simulink model "GFM_Controller_C"  (R2025b)
settings: Solver=VariableStepAuto  StartTime=0.0  StopTime=10.0  RelTol=1e-3
values from neighbouring files (symbols this model uses):
  a = 0.5    [GFM_Simulink_Init_GUI_v3.m]
  b = (beta*gamma)/(beta + gamma - a)    [GFM_Simulink_Init_GUI_v3.m]
  c = (beta + gamma - a)/mp    [GFM_Simulink_Init_GUI_v3.m]
  D1 = Moh_Dp/Moh_Sbase    (= 0.2546)    [GFM_Simulink_Init_GUI_v3.m]
  D2 = 0.4    [GFM_Simulink_Init_GUI_v3.m]
  delta2_0 = delta2PCC0 + atan2(      Pm2_0*X2/V2PCCmag0,      V2PCCmag0 + Q21_0*X2/V2PCCmag0 )    [GFM_Simulink_Init_GUI_v3.m]
  Dw2_0 = 0    [GFM_Simulink_Init_GUI_v3.m]
  E2_0 = hypot(      Pm2_0*X2/V2PCCmag0,      V2PCCmag0 + Q21_0*X2/V2PCCmag0 )    [GFM_Simulink_Init_GUI_v3.m]
  H2 = 12    [GFM_Simulink_Init_GUI_v3.m]
  Imax = 1.20    (= 1.2)    [GFM_Simulink_Init_GUI_v3.m]
  Ki = 0.5    [GFM_Simulink_Init_GUI_v3.m]
  Kiq = Moh_Kiq*Moh_Sbase/Moh_Vbase    [GFM_Simulink_Init_GUI_v3.m]
  Lf = 1e-3    (= 0.001)    [GFM_Simulink_Init_GUI_v3.m]
  LimitEnable = 0    [GFM_Simulink_Init_GUI_v3.m]
  Ls = Xs/ws    [GFM_Simulink_Init_GUI_v3.m]
  nq = Moh_nq*Moh_Sbase/Moh_Vbase    [GFM_Simulink_Init_GUI_v3.m]
  Pload_0 = P12_0    (= 1)    [GFM_Simulink_Init_GUI_v3.m]
  Qref = 0.0    (= 0)    [GFM_Simulink_Init_GUI_v3.m]
  Rf = 1.0    (= 1)    [GFM_Simulink_Init_GUI_v3.m]
  RLFault = 0    [GFM_Simulink_Init_GUI_v3.m]
  Rs = Zs_mag/sqrt(1 + XR_grid^2)    [GFM_Simulink_Init_GUI_v3.m]
  SolidFault = 0    [GFM_Simulink_Init_GUI_v3.m]
  ws = 2*pi*f    (= 314.159265359)    [GFM_Simulink_Init_GUI_v3.m]
  X1 = Xtf_src_total_pu    (= 0.15)    [GFM_Simulink_Init_GUI_v3.m]
libraries: nesl_utility x12, ee_lib x11, fl_lib x6, eePowerMeasurement x1
settings Model: Creator=Nicholas  LastModifiedBy=Nicholas

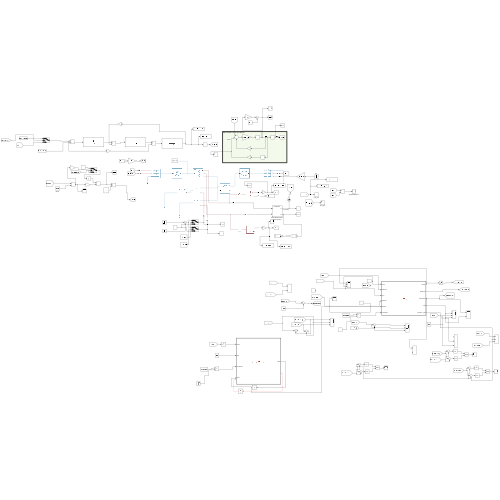
[thumbnail: Simulink's stored preview of the top-level diagram]
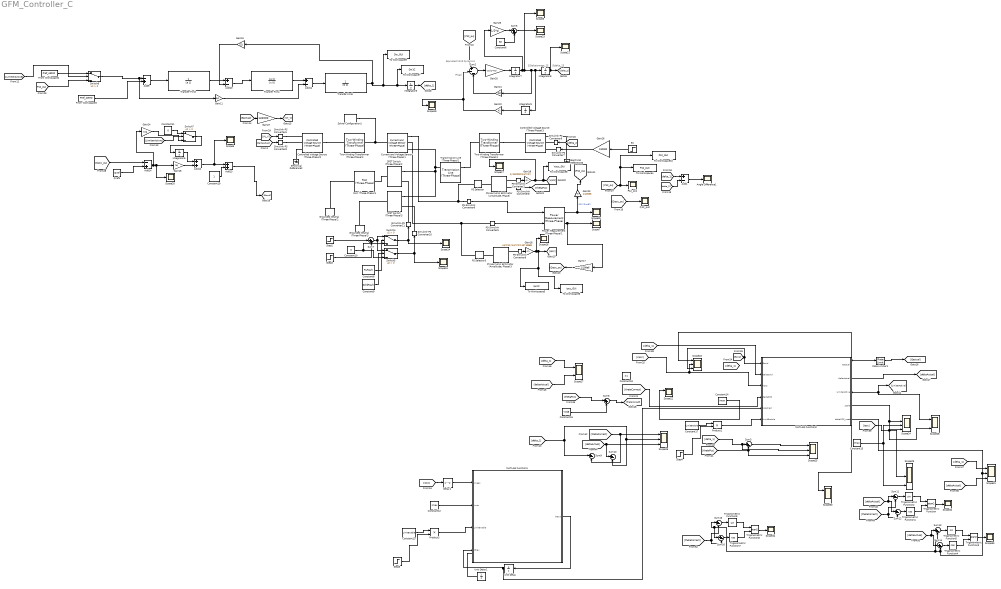
== system GFM_Controller_C ==
  note: $\delta_2$
  note: Pload
  note: $\Delta\omega_2$
  note: Equivalent Grid Dynamics
  Add1 : Sum  Inputs=+-
  Add10 : Sum  Inputs=+-
  Add11 : Sum  Inputs=+-
  Add12 : Sum
  Add13 : Sum
  Add14 : Sum  Inputs=-+
  Add9 : Sum  Inputs=-+
  Angle Difference1 : Scope
      settings: ActiveDisplayYMinimum=-1797.079300536021  ActiveDisplayYMaximum=1392.8706624711849
  Constant10 : Constant  Value=0
  Constant11 : Constant  Value=0
  Constant12 : Constant  Value=Imax
  Constant13 : Constant  Value=LimitEnable
  Constant14 : Constant  Value=Imax
  Constant15 : Constant  Value=Imax
  Constant16 : Constant  Value=-0.58
  Constant17 : Constant  Value=LimitEnable
  Constant18 : Constant  Value=X1
  Constant19 : Constant
  Constant6 : Constant  Value=50
  Constant8 : Constant  Value=RLFault
  Constant9 : Constant  Value=SolidFault
  Controlled Voltage Source (Three-Phase)2 : ee_lib/Sources/Controlled Voltage Source (Three-Phase)  input_option=ee.enum.inputType.singleFreqAC  FRated=50 Hz
      settings: InternalSimscapePortConfiguration="{\"Bottom\":[],\"Left\":[{\"id\":\"Vt\",\"label\":\"Vt\",\"type\":\"input\"},{\"id\":\"ph\",\"label\":\"ph\",\"type\":\"input\"},{\"id\":\"n\",\"label\":\"n\",\"type\":\"foundation.electrical.electrical\"}],\"Right\":[{\"id\":\"N\",\"label\":\"~\",\"type\":\"foundation.electrical.three_phase\"}],\"Top\":[]}"
  Controlled Voltage Source (Three-Phase)3 : ee_lib/Sources/Controlled Voltage Source (Three-Phase)  input_option=ee.enum.inputType.singleFreqAC  FRated=50 Hz
      settings: InternalSimscapePortConfiguration="{\"Bottom\":[],\"Left\":[{\"id\":\"Vt\",\"label\":\"Vt\",\"type\":\"input\"},{\"id\":\"ph\",\"label\":\"ph\",\"type\":\"input\"},{\"id\":\"n\",\"label\":\"n\",\"type\":\"foundation.electrical.electrical\"}],\"Right\":[{\"id\":\"N\",\"label\":\"~\",\"type\":\"foundation.electrical.three_phase\"}],\"Top\":[]}"
  Current and Voltage Sensor (Three-Phase)1 : ee_lib/Sensors & Transducers/Current and Voltage Sensor (Three-Phase)  vMeasurementType=ee.enum.vmeasurement.ll  outputUnit=ee.enum.unit.si  SRated=100e6 A*V  VRated=24e3 V  I_specify=off  I_priority=None  I=[0, 0, 0] A  I_nominal_specify=off  I_nominal_value=1  I_nominal_unit=A  V_specify=off  V_priority=None  V=[0, 0, 0] V  V_nominal_specify=off  V_nominal_value=1  V_nominal_unit=V
      settings: InternalSimscapePortConfiguration="{\"Bottom\":[],\"Left\":[{\"id\":\"N1\",\"label\":\"~1\",\"type\":\"foundation.electrical.three_phase\"}],\"Right\":[{\"id\":\"V_output\",\"label\":\"V\",\"type\":\"output\"},{\"id\":\"I_output\",\"label\":\"I\",\"type\":\"output\"},{\"id\":\"N2\",\"label\":\"~2\",\"type\":\"foundation.electrical.three_phase\"}],\"Top\":[]}"
  Delay1 : Delay  InitialCondition=1  SampleTime=1e-4
  E1 : Step  Before=E2_0  After=E2_0  SampleTime=0
  Electrical Reference2 : fl_lib/Electrical/Electrical Elements/Electrical Reference
  Electrical Reference3 : fl_lib/Electrical/Electrical Elements/Electrical Reference
  From Workspace2 : FromWorkspace  VariableName=Pref_AEMO  Interpolate=off  OutputAfterFinalValue=Holding final value
  From Workspace3 : FromWorkspace  VariableName=Pref_AEMO  Interpolate=off  OutputAfterFinalValue=Holding final value
  Gain11 : Gain  Gain=a/c
  Gain15 : Gain  Gain=D1
  Gain16 : Gain  Gain=nq
  Gain17 : Gain  Gain=1/100e6
  Gain18 : Gain  Gain=sqrt(3)/(sqrt(2)*437.3866)
  Gain19 : Gain  Gain=1/(132000*sqrt(2))
  Gain20 : Gain  Gain=ws/(2*H2)
  Gain21 : Gain  Gain=D2
  Gain22 : Gain  Gain=Ki
  Gain23 : Gain  Gain=1/100e6
  Gain24 : Gain  Gain=Kiq
  Gain25 : Gain  Gain=1/2*pi
  Gain26 : Gain  Gain=132000
  Gain27 : Gain  Gain=132000
  Grounded Neutral (Three-Phase)2 : ee_lib/Connectors & References/Grounded Neutral (Three-Phase)
  Grounded Neutral (Three-Phase)3 : ee_lib/Connectors & References/Grounded Neutral (Three-Phase)
  Integrator5 : Integrator
  Integrator6 : Integrator
  Integrator7 : Integrator  InitialCondition=Dw2_0
  Integrator8 : Integrator  InitialCondition=delta2_0
  Integrator9 : Integrator  InitialCondition=Pload_0/Ki
  MATLAB Function1 : MATLAB Function  TreatAsAtomicUnit=on
  MATLAB Function2 : MATLAB Function  TreatAsAtomicUnit=on
  P12_pu1 : Scope
      settings: ActiveDisplayYMinimum=-0.66145007814127121  ActiveDisplayYMaximum=1.5112363078161035  DataLoggingVariableName=ScopeData4
  "PS Harmonic Estimator (Amplitude, Phase)" : fl_lib/Physical Signals/Periodic Operators/PS Harmonic Estimator (Amplitude, Phase)  f0=50 Hz  n=1  amplMin=0.001 V
      settings: InternalSimscapePortConfiguration="{\"Bottom\":[],\"Left\":[{\"id\":\"I\",\"label\":\"I\",\"type\":\"input\"}],\"Right\":[{\"id\":\"A\",\"label\":\"A\",\"type\":\"output\"},{\"id\":\"Phi\",\"label\":\"Phi\",\"type\":\"output\"}],\"Top\":[]}"
  "PS Harmonic Estimator (Amplitude, Phase)3" : fl_lib/Physical Signals/Periodic Operators/PS Harmonic Estimator (Amplitude, Phase)  f0=50 Hz  n=1  amplMin=0.001 A
      settings: InternalSimscapePortConfiguration="{\"Bottom\":[],\"Left\":[{\"id\":\"I\",\"label\":\"I\",\"type\":\"input\"}],\"Right\":[{\"id\":\"A\",\"label\":\"A\",\"type\":\"output\"},{\"id\":\"Phi\",\"label\":\"Phi\",\"type\":\"output\"}],\"Top\":[]}"
  PS Selector : fl_lib/Physical Signals/Nonlinear Operators/PS Selector  ix=1
      settings: InternalSimscapePortConfiguration="{\"Bottom\":[],\"Left\":[{\"id\":\"I\",\"label\":\"\",\"type\":\"input\"}],\"Right\":[{\"id\":\"O\",\"label\":\"\",\"type\":\"output\"}],\"Top\":[]}"
  PS Selector3 : fl_lib/Physical Signals/Nonlinear Operators/PS Selector  ix=1
      settings: InternalSimscapePortConfiguration="{\"Bottom\":[],\"Left\":[{\"id\":\"I\",\"label\":\"\",\"type\":\"input\"}],\"Right\":[{\"id\":\"O\",\"label\":\"\",\"type\":\"output\"}],\"Top\":[]}"
  PS-Simulink Converter{5..9} (5 alike) : nesl_utility/PS-Simulink Converter  PhysicalDomain=network_engine_domain  SubClassName=ps_output  LeftPortType=input  RightPortType=output  PseudoPeriodic=off  Frequencies=[]  VectorFormat=inherit  Unit=inherit  AffineConversion=off
  Power Measurement (Three-Phase)1 : eePowerMeasurement/Power Measurement (Three-Phase)  LabelModeActiveChoice=Continuous  F=50  K=1  Seq=Positive  Ts=0
  Product1 : Product
  Product3 : Product
  Q12_pu2 : Scope
      settings: ActiveDisplayYMinimum=-2.1630239183901119  ActiveDisplayYMaximum=3.4315471744334132  DataLoggingVariableName=ScopeData5
  Qref1 : Constant  Value=Qref
  RLC (Three-Phase)1 : ee_lib/Passive/RLC Assemblies/RLC (Three-Phase)  port_option=ee.enum.threePhasePort.composite  component_structure=ee.enum.rlc.structure.SeriesRL  R=Rf Ohm  L=Lf H  C=1e-6 F  R_parasitic=0 Ohm  G_parasitic=0 1/Ohm  IL_specify=off  IL_priority=High  IL=[0, 0, 0] A  IL_nominal_specify=off  IL_nominal_value=1  IL_nominal_unit=A  VC_specify=off  VC_priority=High  VC=[0, 0, 0] V  VC_nominal_specify=off  VC_nominal_value=1  VC_nominal_unit=V
      settings: InternalSimscapePortConfiguration="{\"Bottom\":[],\"Left\":[{\"id\":\"N1\",\"label\":\"~1\",\"type\":\"foundation.electrical.three_phase\"}],\"Right\":[{\"id\":\"N2\",\"label\":\"~2\",\"type\":\"foundation.electrical.three_phase\"}],\"Top\":[]}"
  Rate Limiter1 : RateLimiter  RisingSlewLimit=5  FallingSlewLimit=-1000  SampleTimeMode=inherited
  SPST Switch (Three-Phase)2 : ee_lib/Switches & Breakers/SPST Switch (Three-Phase)  R_closed=0.001 Ohm  G_open=1e-6 1/Ohm  threshold=0.5 V  i_vT_specify=off  i_vT_priority=None  i_vT=0 A  i_vT_nominal_specify=off  i_vT_nominal_value=1  i_vT_nominal_unit=A  I_specify=off  I_priority=None  I=[0, 0, 0] A  I_nominal_specify=off  I_nominal_value=1  I_nominal_unit=A  V_specify=off  V_priority=None  V=[0, 0, 0] V  V_nominal_specify=off  V_nominal_value=1  V_nominal_unit=V  i_a_specify=off  i_a_priority=None  i_a=0 A  i_a_nominal_specify=off  i_a_nominal_value=1  i_a_nominal_unit=A  v_a_specify=off  v_a_priority=None  v_a=0 V  v_a_nominal_specify=off  v_a_nominal_value=1  v_a_nominal_unit=V  i_b_specify=off  i_b_priority=None  i_b=0 A  i_b_nominal_specify=off  i_b_nominal_value=1  i_b_nominal_unit=A  v_b_specify=off  v_b_priority=None  v_b=0 V  v_b_nominal_specify=off  v_b_nominal_value=1  v_b_nominal_unit=V  i_c_specify=off  i_c_priority=None  i_c=0 A  i_c_nominal_specify=off  i_c_nominal_value=1  i_c_nominal_unit=A  v_c_specify=off  v_c_priority=None  v_c=0 V  v_c_nominal_specify=off  v_c_nominal_value=1  v_c_nominal_unit=V
      settings: InternalSimscapePortConfiguration="{\"Bottom\":[],\"Left\":[{\"id\":\"vT\",\"label\":\"vT\",\"type\":\"input\"},{\"id\":\"N1\",\"label\":\"~1\",\"type\":\"foundation.electrical.three_phase\"}],\"Right\":[{\"id\":\"N2\",\"label\":\"~2\",\"type\":\"foundation.electrical.three_phase\"}],\"Top\":[]}"
  SPST Switch (Three-Phase)3 : ee_lib/Switches & Breakers/SPST Switch (Three-Phase)  R_closed=0.001 Ohm  G_open=1e-6 1/Ohm  threshold=0.5 V  i_vT_specify=off  i_vT_priority=None  i_vT=0 A  i_vT_nominal_specify=off  i_vT_nominal_value=1  i_vT_nominal_unit=A  I_specify=off  I_priority=None  I=[0, 0, 0] A  I_nominal_specify=off  I_nominal_value=1  I_nominal_unit=A  V_specify=off  V_priority=None  V=[0, 0, 0] V  V_nominal_specify=off  V_nominal_value=1  V_nominal_unit=V  i_a_specify=off  i_a_priority=None  i_a=0 A  i_a_nominal_specify=off  i_a_nominal_value=1  i_a_nominal_unit=A  v_a_specify=off  v_a_priority=None  v_a=0 V  v_a_nominal_specify=off  v_a_nominal_value=1  v_a_nominal_unit=V  i_b_specify=off  i_b_priority=None  i_b=0 A  i_b_nominal_specify=off  i_b_nominal_value=1  i_b_nominal_unit=A  v_b_specify=off  v_b_priority=None  v_b=0 V  v_b_nominal_specify=off  v_b_nominal_value=1  v_b_nominal_unit=V  i_c_specify=off  i_c_priority=None  i_c=0 A  i_c_nominal_specify=off  i_c_nominal_value=1  i_c_nominal_unit=A  v_c_specify=off  v_c_priority=None  v_c=0 V  v_c_nominal_specify=off  v_c_nominal_value=1  v_c_nominal_unit=V
      settings: InternalSimscapePortConfiguration="{\"Bottom\":[],\"Left\":[{\"id\":\"vT\",\"label\":\"vT\",\"type\":\"input\"},{\"id\":\"N1\",\"label\":\"~1\",\"type\":\"foundation.electrical.three_phase\"}],\"Right\":[{\"id\":\"N2\",\"label\":\"~2\",\"type\":\"foundation.electrical.three_phase\"}],\"Top\":[]}"
  Scope{3,5,7,14..17,19..21,23,32..35} (15 alike) : Scope
      Scope14 settings: ActiveDisplayYMinimum=-1  ActiveDisplayYMaximum=1  DataLoggingVariableName=ScopeData7
      Scope15 settings: ActiveDisplayYMinimum=-1  ActiveDisplayYMaximum=1  DataLoggingVariableName=ScopeData16
      Scope16 settings: ActiveDisplayYMinimum=-1.0313612715858387  ActiveDisplayYMaximum=9.28225144427255  DataLoggingVariableName=ScopeData17
      Scope17 settings: ActiveDisplayYMinimum=-2.5658886223026931  ActiveDisplayYMaximum=3.94553749363296  DataLoggingVariableName=ScopeData48
      Scope19 settings: ActiveDisplayYMinimum=-1.1623447136135812  ActiveDisplayYMaximum=1.3781315704633705  DataLoggingVariableName=ScopeData19
      Scope20 settings: ActiveDisplayYMinimum=-1.22917  ActiveDisplayYMaximum=1.0625  DataLoggingVariableName=ScopeData21
      Scope21 settings: DataLoggingVariableName=ScopeData23
      Scope23 settings: ActiveDisplayYMinimum=49.92788610274394  ActiveDisplayYMaximum=50.170097472488152  DataLoggingVariableName=ScopeData24
      Scope3 settings: DataLoggingVariableName=ScopeData25
      Scope32 settings: ActiveDisplayYMinimum=-3.9269892876580919  ActiveDisplayYMaximum=3.9269891159141448  DataLoggingVariableName=ScopeData78
      Scope33 settings: ActiveDisplayYMinimum=-1  ActiveDisplayYMaximum=1  DataLoggingVariableName=ScopeData79
      Scope34 settings: ActiveDisplayYMinimum=-1.4401977699145856  ActiveDisplayYMaximum=2.6200072427590877  DataLoggingVariableName=ScopeData80
      Scope35 settings: ActiveDisplayYMinimum=-1.1115259938999555E+8  ActiveDisplayYMaximum=2.0473695052149418E+8  DataLoggingVariableName=ScopeData27
      Scope5 settings: ActiveDisplayYMinimum=-0.05189  ActiveDisplayYMaximum=0.00577  DataLoggingVariableName=ScopeData28
      Scope7 settings: ActiveDisplayYMinimum=-7.0875379074731711E+6  ActiveDisplayYMaximum=3.5866343126415364E+7  DataLoggingVariableName=ScopeData29
  Scope{18,25..26,29,31} (5 alike) : Scope  NumInputPorts=3
      Scope18 settings: ActiveDisplayYMinimum=-0.12862546618818504  ActiveDisplayYMaximum=1.1576291956936657  DataLoggingVariableName=ScopeData18
      Scope25 settings: ActiveDisplayYMinimum=-2.6035343832796971  ActiveDisplayYMaximum=9.8526279409331341  DataLoggingVariableName=ScopeData71
      Scope26 settings: ActiveDisplayYMinimum=-2.7720251649113785  ActiveDisplayYMaximum=1.647845241487004  DataLoggingVariableName=ScopeData72
      Scope29 settings: ActiveDisplayYMinimum=-0.5707391589619073  ActiveDisplayYMaximum=5.1366524306571666  DataLoggingVariableName=ScopeData75
      Scope31 settings: ActiveDisplayYMinimum=-2.7504004579249388  ActiveDisplayYMaximum=0.52931298913436242  DataLoggingVariableName=ScopeData77
  Scope{22,27..28,30} (4 alike) : Scope  NumInputPorts=2
      Scope22 settings: ActiveDisplayYMinimum=-1.1863011737345548  ActiveDisplayYMaximum=10.676710563610996  DataLoggingVariableName=ScopeData81
      Scope27 settings: ActiveDisplayYMinimum=-3.7225747393161841  ActiveDisplayYMaximum=4.13168438536474  DataLoggingVariableName=ScopeData73
      Scope28 settings: ActiveDisplayYMinimum=-0.12499999999999997  ActiveDisplayYMaximum=1.125  DataLoggingVariableName=ScopeData74
      Scope30 settings: ActiveDisplayYMinimum=-0.12499999999999997  ActiveDisplayYMaximum=1.125  DataLoggingVariableName=ScopeData76
  Scope24 : Scope  NumInputPorts=4
      settings: ActiveDisplayYMinimum=-1.1228736312304088  ActiveDisplayYMaximum=10.105862681073681  DataLoggingVariableName=ScopeData26
  Simulink-PS Converter{6..11} (6 alike) : nesl_utility/Simulink-PS Converter  PhysicalDomain=network_engine_domain  SubClassName=ps_input  LeftPortType=input  RightPortType=output  PseudoPeriodic=off  Frequencies=[]  NoiseDistribution=none  NoiseParameters=[]  Unit=1  AffineConversion=off  FilteringAndDerivatives=provide  SimscapeFilterOrder=1  InputFilterTimeConstant=0.001  UdotUserProvided=0
  Solver Configuration1 : nesl_utility/Solver Configuration  PhysicalDomain=network_engine_domain  SubClassName=solver  LeftPortType=input  RightPortType=generic  Tones=[]  Harmonics=[]  SimulateNoise=off  Profile=off  UseLocalSampling=off  EnableSwitchedLinearOptims=on  FrequencyDomain=off  UseCCode=off  RelTol=0.001  AbsTol=0.001  MinStep=1e-09  ToWorkspace=off  RevertToSquareIcSolve=off  NumHomotopyIterations=100  PhasorMode=off  PhasorModeNumHarmonics=1  ConsistencySolver=NEWTON_XTOL_AFTER_FTOL  IndexReductionMethod=DerivativeReplacement  DoDC=off  ResidualTolerance=1e-09  ConsistencyTolSource=GLOBAL  ConsistencyAbsTol=0.001  ConsistencyRelTol=0.001  ConsistencyTolFactor=0.001  UseLocalSolver=off  LocalSolverChoice=NE_BACKWARD_EULER_ADVANCER  ResolveIndetEquations=on  FunctionEvalNumThread=1  LocalSolverSampleTime=0.001  DoFixedCost=off  MaxNonlinIter=3  MaxModeIter=2  ComputeImpulses=off  ImpulseIterations=2  LinearAlgebra=auto  LinearAlgebraNumThread=0  EquationFormulation=NE_TIME_EF  DelaysMemoryBudget=16384  AutomaticFiltering=on  FilteringTimeConstant=0.001  PartitionStorageMethod=AS_NEEDED  PartitionMemoryBudget=1024  PartitionMethod=ROBUST  MultibodyUseLocalSolver=off  MultibodyLocalSolverChoice=ODE1  MultibodyLocalSolverSampleTime=0.001
  Step2 : Step  Time=5  SampleTime=0
  Step3 : Step  Time=5.43  After=-1  SampleTime=0
  Step4 : Step  Time=3  SampleTime=0
  Step5 : Step  Time=3  SampleTime=0
  Sum{3,9..16} (9 alike) : Sum  Inputs=|+-
  Sum2 : Sum  Inputs=|+|-|-
  Sum5 : Sum  Inputs=|++
  Sum7 : Sum  Inputs=|++
  Sum8 : Sum  Inputs=|++
  Switch{4..7} (4 alike) : Switch  Criteria=u2 > Threshold  SaturateOnIntegerOverflow=off  InputSameDT=off
  To Workspace10 : ToWorkspace  VariableName=P12_GUI  SaveFormat=Timeseries  SampleTime=-1
  To Workspace4 : ToWorkspace  VariableName=P12_puC  SaveFormat=Timeseries  SampleTime=-1
  To Workspace5 : ToWorkspace  VariableName=IpccC  SaveFormat=Timeseries  SampleTime=-1
  To Workspace6 : ToWorkspace  VariableName=Ipcc_GUI  SaveFormat=Timeseries  SampleTime=-1
  To Workspace7 : ToWorkspace  VariableName=Dw1C  SaveFormat=Timeseries  SampleTime=-1
  To Workspace8 : ToWorkspace  VariableName=Vpcc_GUI  SaveFormat=Timeseries  SampleTime=-1
  To Workspace9 : ToWorkspace  VariableName=Dw_GUI  SaveFormat=Timeseries  SampleTime=-1
  Transfer Fcn3 : TransferFcn  Denominator=[a 1]
  Transfer Fcn4 : TransferFcn  Numerator=[a 1]  Denominator=[c 0]
  Transfer Fcn5 : TransferFcn  Denominator=[b 1]
  Transmission Line (Three-Phase)1 : ee_lib/Passive/Lines/Transmission Line (Three-Phase)  length=1 km  freq=f Hz  R=Rs Ohm/km  L=Ls*1000 mH/km  M=0 mH/km  Cl=0.3 uF/km  Cg=0.1 uF/km  Rm=0 Ohm/km  ModelTwoSections=ee.enum.enable.no  N=1  InterfacePosition=0.5 km  N1sec=1  N2sec=1  Access_ground=ee.enum.enable.no  R_parasitic=1e-6 Ohm  G_parasitic=1e-6 1/Ohm
      settings: InternalSimscapePortConfiguration="{\"Bottom\":[],\"Left\":[{\"id\":\"N1\",\"label\":\"~1\",\"type\":\"foundation.electrical.three_phase\"},{\"id\":\"g1\",\"label\":\"g1\",\"type\":\"foundation.electrical.electrical\"}],\"Right\":[{\"id\":\"N2\",\"label\":\"~2\",\"type\":\"foundation.electrical.three_phase\"},{\"id\":\"g2\",\"label\":\"g2\",\"type\":\"foundation.electrical.electrical\"}],\"Top\":[]}"
  Trigonometric Function : Trigonometry  Operator=atan2
  Trigonometric Function1 : Trigonometry  Operator=cos
  Trigonometric Function2 : Trigonometry
  Trigonometric Function3 : Trigonometry  Operator=atan2
  Trigonometric Function4 : Trigonometry  Operator=cos
  Trigonometric Function5 : Trigonometry
  Trigonometric Function6 : Trigonometry  Operator=atan2
  Trigonometric Function7 : Trigonometry  Operator=cos
  Trigonometric Function8 : Trigonometry
  Two-Winding Transformer (Three-Phase)2 : ee_lib/Passive/Transformers/Two-Winding Transformer (Three-Phase)  SRated=100e6 A*V  FRated=50 Hz  Winding1Connection=ee.enum.windingconnection.Yg  VRated1=132000 V  Winding2Connection=ee.enum.windingconnection.Yg  VRated2=132000 V  CoreType=ee.enum.coretype.threelimb  pu_Rw1=0.001  pu_Rw2=0.001  leakage_reactance_option=ee.enum.transformer_leakage.include  pu_Xl1=0.075  pu_Xl2=0.075  magnetizing_resistance_option=ee.enum.transformer_magnetizingResistance.exclude  pu_Rm=500  magnetizing_reactance_option=ee.enum.transformer_magnetizingReactance.exclude  saturation_option=ee.enum.transformer_saturation.exclude  pu_Xm=500  current_data=[0, .002, 1, 2]  magnetic_flux_data=[0, 1.2, 1.5, 1.51]  pu_X0=0.5  i1_specify=off  i1_priority=None  i1=[0, 0, 0] A  i1_nominal_specify=off  i1_nominal_value=1  i1_nominal_unit=A  i2_specify=off  i2_priority=None  i2=[0, 0, 0] A  i2_nominal_specify=off  i2_nominal_value=1  i2_nominal_unit=A  phi_specify=off  phi_priority=None  phi=[0, 0, 0]  phi_nominal_specify=off  phi_nominal_value=1  phi_nominal_unit=1  power_dissipated_specify=off  power_dissipated_priority=None  power_dissipated=0 W  power_dissipated_nominal_specify=off  power_dissipated_nominal_value=1  power_dissipated_nominal_unit=W
      settings: InternalSimscapePortConfiguration="{\"Bottom\":[],\"Left\":[{\"id\":\"N1\",\"label\":\"~1\",\"type\":\"foundation.electrical.three_phase\"}],\"Right\":[{\"id\":\"N2\",\"label\":\"~2\",\"type\":\"foundation.electrical.three_phase\"}],\"Top\":[]}"
  Two-Winding Transformer (Three-Phase)3 : ee_lib/Passive/Transformers/Two-Winding Transformer (Three-Phase)  SRated=100e6 A*V  FRated=50 Hz  Winding1Connection=ee.enum.windingconnection.Y  VRated1=132000 V  Winding2Connection=ee.enum.windingconnection.Y  VRated2=132000 V  CoreType=ee.enum.coretype.threelimb  pu_Rw1=0.001  pu_Rw2=0.001  leakage_reactance_option=ee.enum.transformer_leakage.include  pu_Xl1=0.075  pu_Xl2=0.075  magnetizing_resistance_option=ee.enum.transformer_magnetizingResistance.exclude  pu_Rm=500  magnetizing_reactance_option=ee.enum.transformer_magnetizingReactance.exclude  saturation_option=ee.enum.transformer_saturation.exclude  pu_Xm=500  current_data=[0, .002, 1, 2]  magnetic_flux_data=[0, 1.2, 1.5, 1.51]  pu_X0=0.5  i1_specify=off  i1_priority=None  i1=[0, 0, 0] A  i1_nominal_specify=off  i1_nominal_value=1  i1_nominal_unit=A  i2_specify=off  i2_priority=None  i2=[0, 0, 0] A  i2_nominal_specify=off  i2_nominal_value=1  i2_nominal_unit=A  phi_specify=off  phi_priority=None  phi=[0, 0, 0]  phi_nominal_specify=off  phi_nominal_value=1  phi_nominal_unit=1  power_dissipated_specify=off  power_dissipated_priority=None  power_dissipated=0 W  power_dissipated_nominal_specify=off  power_dissipated_nominal_value=1  power_dissipated_nominal_unit=W
      settings: InternalSimscapePortConfiguration="{\"Bottom\":[],\"Left\":[{\"id\":\"N1\",\"label\":\"~1\",\"type\":\"foundation.electrical.three_phase\"}],\"Right\":[{\"id\":\"N2\",\"label\":\"~2\",\"type\":\"foundation.electrical.three_phase\"}],\"Top\":[]}"
  Unit Delay : UnitDelay  InitialCondition=1  SampleTime=1e-4  HasFrameUpgradeWarning=on
  Unit Delay1 : UnitDelay  InitialCondition=1  SampleTime=1e-4  HasFrameUpgradeWarning=on
  wires:
  Gain18/1 -> To Workspace6/1, To Workspace5/1, [Ipcc], Scope16/1
  Add14/1 -> Gain24/1, Scope20/1, Gain16/1
  Gain11/1 -> Add11/2
  Constant8/1 -> Switch4/2
  Sum5/1 -> Scope23/1
  Add11/1 -> Transfer Fcn5/1
  [thetaCorrect] -> Sum16/2, Sum15/2
  Sum15/1 -> Trigonometric Function8/1
  Power Measurement (Three-Phase)1/2 -> Scope7/1, Gain17/1
  [P12_pu] -> To Workspace10/1, To Workspace4/1, P12_pu1/1
  Gain25/1 -> Sum5/1
  [thetaCorrect] -> Sum9/2, Scope26/1
  Switch5/1 -> Scope15/1, Simulink-PS Converter10/1
  [Vt_V] -> Simulink-PS Converter6/1
  [Vpcc] -> Scope18/2, MATLAB Function2/3(Vpcc)
  Rate Limiter1/1 -> [Eactual]
  Constant19/1 -> Add13/2
  [P12_pu] -> Sum2/1
  MATLAB Function2/5(deltaPCC_used) -> Sum13/2, Sum15/1, Sum16/1, Sum14/2, Scope31/2
  Gain15/1 -> Add10/2
  Add1/1 -> Angle Difference1/1
  Constant17/1 -> Product1/1
  Sum16/1 -> Trigonometric Function7/1
  Gain27/1 -> [Vt_V]
  Trigonometric Function3/1 -> Scope33/1
  [delta_2] -> Simulink-PS Converter9/1
  Gain16/1 -> Add12/2
  Sum12/1 -> Trigonometric Function1/1
  Integrator5/1 -> [delta_1]
  E1/1 -> Gain26/1
  [deltaActual] -> Sum14/1, Sum13/1
  Add9/1 -> Transfer Fcn3/1
  Trigonometric Function6/1 -> Scope34/1
  [delta_1] -> Add1/1
  From Workspace3/1 -> Add9/2
  Sum14/1 -> Trigonometric Function4/1
  Trigonometric Function2/1 -> Trigonometric Function/1
  Gain24/1 -> Switch7/3
  Integrator9/1 -> Gain22/1
  [Ipcc] -> Delay1/1
  PS-Simulink Converter5/1 -> Power Measurement (Three-Phase)1/2
  Integrator6/1 -> Add12/1
  Sum2/1 -> Gain20/1
  [deltaActual] -> Scope31/3
  Trigonometric Function1/1 -> Trigonometric Function/2
  [delta_1] -> Scope27/1
  [delta_1] -> Sum9/1, Sum10/2, Scope26/2
  Add10/1 -> Transfer Fcn4/1
  Gain20/1 -> Integrator7/1
  Switch7/1 -> Integrator6/1
  Constant15/1 -> Scope29/3, Scope24/3
  Power Measurement (Three-Phase)1/1 -> Scope35/1, Gain23/1  "P12 (SimEl)"
  [thetaPcc] -> Sum8/1
  [Eactual] -> Gain27/1
  Transfer Fcn5/1 -> To Workspace9/1, To Workspace7/1, Integrator5/1, Gain15/1
  [Qpcc_pu] -> Q12_pu2/1
  MATLAB Function2/3(LimiterActive) -> Scope30/1, [LimiterActive], Scope28/1
  Transfer Fcn4/1 -> Add11/1
  MATLAB Function2/2(deltaActual) -> [deltaActual]
  Constant10/1 -> Switch5/3, Switch4/3
  Product3/1 -> MATLAB Function1/3(LimitEnable)
  Integrator8/1 -> [delta_2], Scope21/1
  Trigonometric Function5/1 -> Trigonometric Function3/1
  From Workspace2/1 -> Switch6/1
  Step5/1 -> Product3/2
  Sum8/1 -> [thetaCorrect]
  [delta_1] -> MATLAB Function2/2(deltaCmd)
  [P12_pu] -> Switch6/3
  Gain19/1 -> Scope17/1, To Workspace8/1, [Vpcc]
  Constant13/1 -> Product3/1
  [LimiterActive] -> Switch7/2
  Add13/1 -> [Ecmd]
  MATLAB Function2/4(scale) -> Scope28/2, Scope24/2
  [thetaCorrect] -> Sum12/2, Sum11/2
  Constant16/1 -> Sum8/2
  Integrator7/1 -> Gain25/1, Scope3/1, Gain21/1, Integrator9/1, Integrator8/1
  [Qpcc_pu] -> Add14/1
  Sum7/1 -> Switch5/1, Switch4/1
  Gain17/1 -> [Qpcc_pu]
  MATLAB Function2/1(Eactual) -> Scope18/1, Rate Limiter1/1
  Constant6/1 -> Sum5/2
  PS-Simulink Converter9/1 -> Gain18/1
  MATLAB Function1/1(kNext) -> Unit Delay/1
  [Ipcc] -> Scope29/2, Scope24/4
  Unit Delay/1 -> MATLAB Function2/5(kApplied), MATLAB Function1/4(kPrev)
  Gain22/1 -> Scope19/1, Sum2/2
  Trigonometric Function4/1 -> Trigonometric Function3/2
  Step3/1 -> Sum7/2
  [thetaPcc] -> Scope25/3, Sum3/2
  [delta_2] -> Add1/2
  Product1/1 -> MATLAB Function2/6(LimitEnable)
  Transfer Fcn3/1 -> Add10/1
  [delta_1] -> Scope31/1
  Step4/1 -> Product1/2
  Gain23/1 -> [P12_pu]
  Add12/1 -> Scope5/1, Add13/1
  Trigonometric Function/1 -> Scope32/1
  Constant12/1 -> MATLAB Function1/2(Imax)
  Trigonometric Function7/1 -> Trigonometric Function6/2
  [delta_1] -> Scope25/2, Sum3/1
  [thetaCorrect] -> MATLAB Function2/4(deltaPCC)
  Gain21/1 -> Sum2/3
  Switch4/1 -> Simulink-PS Converter11/1, Scope14/1
  [LimiterActive] -> Switch6/2
  PS-Simulink Converter8/1 -> [thetaPcc]
  Sum13/1 -> Trigonometric Function5/1
  PS-Simulink Converter7/1 -> Gain19/1
  Step2/1 -> Sum7/1
  Constant14/1 -> Scope22/1
  [deltaActual] -> Scope27/2
  Gain26/1 -> Simulink-PS Converter7/1
  [deltaActual] -> Sum10/1, Scope26/3
  Switch6/1 -> Gain11/1, Add9/1
  [deltaActual] -> Simulink-PS Converter8/1
  Trigonometric Function8/1 -> Trigonometric Function6/1
  Delay1/1 -> MATLAB Function1/1(Imeas)
  [deltaActual] -> Sum12/1, Sum11/1
  Constant9/1 -> Switch5/2
  [Ecmd] -> Scope18/3, MATLAB Function2/1(Ecmd)
  Sum3/1 -> Scope25/1
  Sum11/1 -> Trigonometric Function2/1
  Constant11/1 -> Switch7/1
  ? -> Unit Delay1/1
  Unit Delay1/1 -> ?
  Qref1/1 -> Add14/2
  PS-Simulink Converter6/1 -> Power Measurement (Three-Phase)1/1
  connections:
  SPST Switch (Three-Phase)3/LConn2 -- SPST Switch (Three-Phase)2/LConn2 -- Current and Voltage Sensor (Three-Phase)1/RConn3 -- Transmission Line (Three-Phase)1/LConn1
  Two-Winding Transformer (Three-Phase)2/RConn1 -- Current and Voltage Sensor (Three-Phase)1/LConn1 -- Solver Configuration1/RConn1
  Current and Voltage Sensor (Three-Phase)1/RConn2 -- PS-Simulink Converter5/LConn1 -- PS Selector3/LConn1
  PS-Simulink Converter6/LConn1 -- Current and Voltage Sensor (Three-Phase)1/RConn1 -- PS Selector/LConn1
  SPST Switch (Three-Phase)2/RConn1 -- RLC (Three-Phase)1/RConn1
  Electrical Reference3/LConn1 -- Controlled Voltage Source (Three-Phase)3/LConn3
  Simulink-PS Converter8/RConn1 -- Controlled Voltage Source (Three-Phase)2/LConn2
  Transmission Line (Three-Phase)1/RConn1 -- Two-Winding Transformer (Three-Phase)3/LConn1
  Grounded Neutral (Three-Phase)2/LConn1 -- RLC (Three-Phase)1/LConn1
  Simulink-PS Converter6/RConn1 -- Controlled Voltage Source (Three-Phase)2/LConn1
  Simulink-PS Converter10/RConn1 -- SPST Switch (Three-Phase)3/LConn1
  Simulink-PS Converter7/RConn1 -- Controlled Voltage Source (Three-Phase)3/LConn1
  "PS Harmonic Estimator (Amplitude, Phase)3"/LConn1 -- PS Selector3/RConn1
  Simulink-PS Converter11/RConn1 -- SPST Switch (Three-Phase)2/LConn1
  PS-Simulink Converter9/LConn1 -- "PS Harmonic Estimator (Amplitude, Phase)3"/RConn1
  Electrical Reference2/LConn1 -- Controlled Voltage Source (Three-Phase)2/LConn3
  "PS Harmonic Estimator (Amplitude, Phase)"/LConn1 -- PS Selector/RConn1
  Simulink-PS Converter9/RConn1 -- Controlled Voltage Source (Three-Phase)3/LConn2
  Controlled Voltage Source (Three-Phase)2/RConn1 -- Two-Winding Transformer (Three-Phase)2/LConn1
  SPST Switch (Three-Phase)3/RConn1 -- Grounded Neutral (Three-Phase)3/LConn1
  PS-Simulink Converter8/LConn1 -- "PS Harmonic Estimator (Amplitude, Phase)"/RConn2
  PS-Simulink Converter7/LConn1 -- "PS Harmonic Estimator (Amplitude, Phase)"/RConn1
  Two-Winding Transformer (Three-Phase)3/RConn1 -- Controlled Voltage Source (Three-Phase)3/RConn1

== matlab function GFM_Controller_C/MATLAB Function1 ==
  data: Imeas input; kNext output; Imax input; LimitEnable input; kPrev input

function kNext = CurrentScaleController(Imeas,Imax,LimitEnable,kPrev)

% Discrete exponential current limiter
% All currents in pu

Ts = 1e-4;          % Sample time [s]

Kdown = 10;         % Current reduction gain
Kup   = 4;          % Recovery gain

Kmin = 0.02;        % Minimum voltage scaling
releaseMargin = 0.05;

Ion  = Imax;
Ioff = max(Imax-releaseMargin,0);

% Disable limiter
if LimitEnable < 0.5
    kNext = 1;
    return;
end

% CURRENT ABOVE LIMIT - exponentially reduce scaling
if Imeas > Ion

    excess = Imeas-Ion;

    kNext = kPrev*exp(-Kdown*excess*Ts);

% CURRENT BELOW RELEASE THRESHOLD - recover gradually
elseif Imeas < Ioff

    kNext = 1-(1-kPrev)*exp(-Kup*Ts);

% CURRENT WITHIN DEADBAND - hold previous scaling
else

    kNext = kPrev;

end

% Bound scaling
kNext = min(1,max(Kmin,kNext));

end

== matlab function GFM_Controller_C/MATLAB Function2 ==
  data: Ecmd input; Eactual output; deltaActual output; deltaCmd input; Vpcc input; deltaPCC input; kApplied input; LimitEnable input; LimiterActive output; scale output; deltaPCC_used output

function [Eactual,deltaActual,LimiterActive,scale,deltaPCC_used] = ...
    CurrentLimiter(Ecmd,deltaCmd,Vpcc,deltaPCC,kApplied,LimitEnable)

% ============================================================
% PHASOR CURRENT LIMITER
%
% Scaling is controlled externally by CurrentScaleController.
%
% Inputs:
% Ecmd        - commanded voltage magnitude [pu]
% deltaCmd    - commanded source angle [rad]
% Vpcc        - measured PCC voltage magnitude [pu]
% deltaPCC    - measured PCC phase angle [rad]
% kApplied    - scaling from external discrete controller
% LimitEnable - limiter enable (0 or 1)
%
% Outputs:
% Eactual       - applied source voltage magnitude [pu]
% deltaActual   - applied source voltage angle [rad]
% LimiterActive - limiter status
% scale         - applied scaling factor
% deltaPCC_used - corrected PCC angle used by limiter
% ============================================================

%% PCC angle settings

thetaOffset   = 0;
deltaThetaRef = 0.15;

Vlow  = 0.20;
Vhigh = 0.80;

%% External current-limiting scale

if LimitEnable > 0.5

    % Use scale generated by CurrentScaleController
    scale = min(1,max(0,kApplied));

else

    % Limiter disabled: full pass-through
    scale = 1;

end

LimiterActive = (LimitEnable > 0.5) && (scale < 0.999);

%% Correct PCC angle reference

deltaPCC_meas = deltaPCC - thetaOffset;

relMeasured = atan2( ...
    sin(deltaPCC_meas - deltaCmd), ...
    cos(deltaPCC_meas - deltaCmd));

%% Low-voltage angle fallback

relFallback = -deltaThetaRef;

%% Smooth low-voltage angle blending

% Voltage-based phase reliability
alphaV = (Vpcc - Vlow)/(Vhigh - Vlow);
alphaV = min(1,max(0,alphaV));

% Suppress PCC phase feedback during strong limiting
alphaK = (scale - 0.80)/0.20;
alphaK = min(1,max(0,alphaK));

% Combined blending factor
alpha = alphaV;

relError = atan2( ...
    sin(relMeasured - relFallback), ...
    cos(relMeasured - relFallback));

relUsed = relFallback + alpha*relError;

deltaPCC_used = deltaCmd + relUsed;

%% Build PCC voltage phasor in local reference

Vpcc_local = Vpcc*exp(1j*relUsed);

%% Apply external scaling to voltage phasor

Eactual_local = ...
    Vpcc_local + scale*(Ecmd - Vpcc_local);

%% Calculate magnitude and phase

Eactual = abs(Eactual_local);

deltaCorrection = angle(Eactual_local);

deltaActual = deltaCmd + deltaCorrection;

%% Exact bypass when limiter is inactive

if scale >= 1

    Eactual = Ecmd;
    deltaActual = deltaCmd;

end

end
